simulink model "Shift_Timer_Test"  (R2023b)
settings: Solver=FixedStepDiscrete  StartTime=0.0  StopTime=160  FixedStep=0.02  RelTol=1e-3
values from neighbouring files (symbols this model uses):
  Rebuilt_Match_Time_Auto_Timer = Auto_Timer - Time_offset    (= 27)    [Shift_Timer_Test_Data.m]
  Rebuilt_Match_Time_End_Game_Timer = End_Game_Timer + Time_offset    (= 33)    [Shift_Timer_Test_Data.m]
  Rebuilt_Match_Time_Shift_1 = Time_Shift_1 - Time_offset    (= 32)    [Shift_Timer_Test_Data.m]
  Rebuilt_Match_Time_Shift_2 = Time_Shift_2 - Time_offset    (= 57)    [Shift_Timer_Test_Data.m]
  Rebuilt_Match_Time_Shift_3 = Time_Shift_3 - Time_offset    (= 82)    [Shift_Timer_Test_Data.m]
  Rebuilt_Match_Time_Shift_4 = Time_Shift_4 - Time_offset    (= 107)    [Shift_Timer_Test_Data.m]
  Rebuilt_Match_Time_Shift_Timer = Shift_Timer    (= 25)    [Shift_Timer_Test_Data.m]
undefined symbols (not defined in the file or in its folder): Rebuilt_Match_Time_Shoot_Early, Rebuilt_Match_Time_Transition, t_sample
libraries: simulink x13
settings Model: Creator=FIRSTMentor  LastModifiedBy=ander

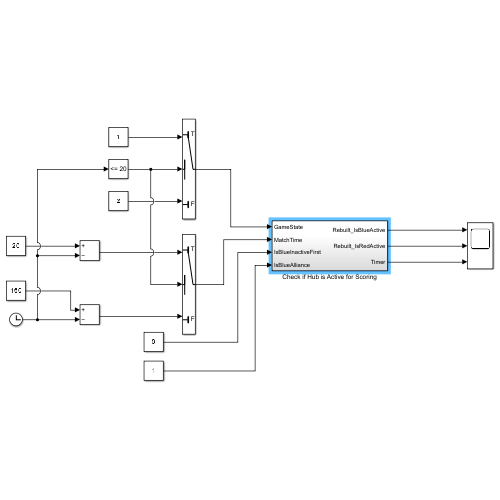
[thumbnail: Simulink's stored preview of the top-level diagram]
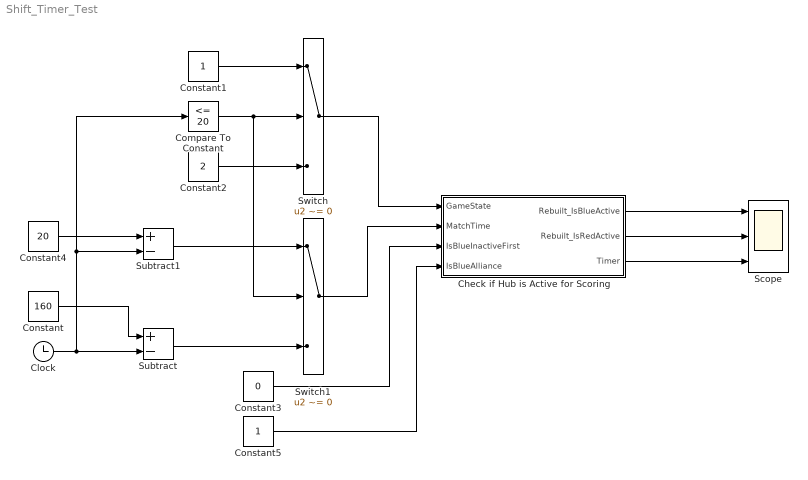
== system Shift_Timer_Test ==
  Check if Hub is Active for Scoring : Subsystem
  Clock : Clock
  Compare To Constant : simulink/Logic and Bit Operations/Compare To Constant  relop=<=  const=20  OutDataTypeStr=boolean
  Constant : Constant  Value=160
  Constant1 : Constant
  Constant2 : Constant  Value=2
  Constant3 : Constant  Value=0  OutDataTypeStr=boolean
  Constant4 : Constant  Value=20
  Constant5 : Constant  OutDataTypeStr=boolean
  Scope : Scope  NumInputPorts=3
  Subtract : Sum  Inputs=+-
  Subtract1 : Sum  Inputs=+-
  Switch : Switch  Criteria=u2 ~= 0  SaturateOnIntegerOverflow=off  InputSameDT=off
  Switch1 : Switch  Criteria=u2 ~= 0  SaturateOnIntegerOverflow=off  InputSameDT=off
  wires:
  Clock/1 -> Subtract/2, Subtract1/2, Compare To Constant/1
  Constant/1 -> Subtract/1
  Compare To Constant/1 -> Switch1/2, Switch/2
  Constant1/1 -> Switch/1
  Constant2/1 -> Switch/3
  Switch/1 -> Check if Hub is Active for Scoring/1(GameState)
  Constant3/1 -> Check if Hub is Active for Scoring/3(IsBlueInactiveFirst)
  Check if Hub is Active for Scoring/1(Rebuilt_IsBlueActive) -> Scope/1
  Check if Hub is Active for Scoring/2(Rebuilt_IsRedActive) -> Scope/2
  Check if Hub is Active for Scoring/3(Timer) -> Scope/3
  Switch1/1 -> Check if Hub is Active for Scoring/2(MatchTime)
  Subtract/1 -> Switch1/3
  Subtract1/1 -> Switch1/1
  Constant4/1 -> Subtract1/1
  Constant5/1 -> Check if Hub is Active for Scoring/4(IsBlueAlliance)

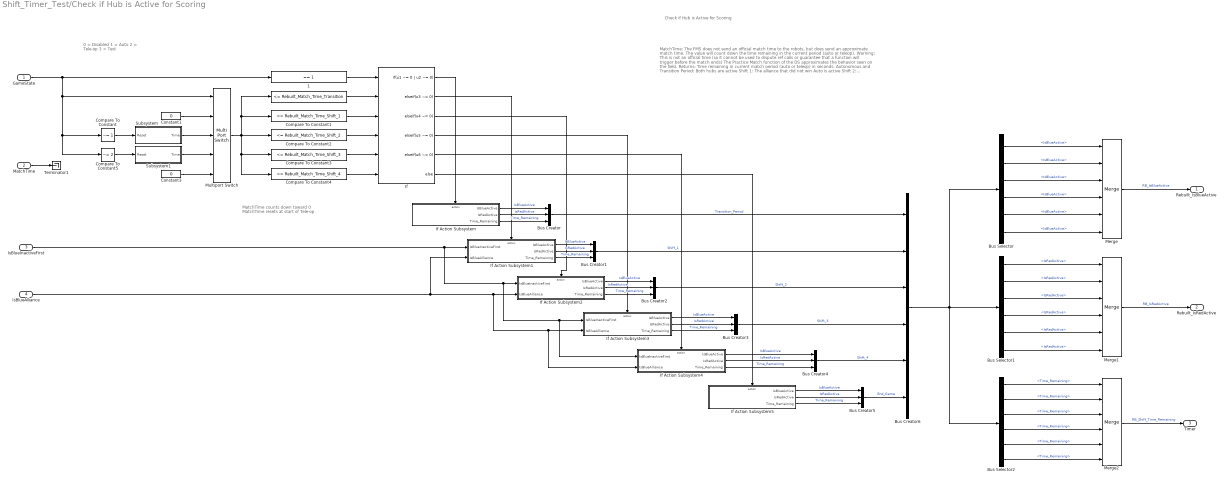
== system Shift_Timer_Test/Check if Hub is Active for Scoring ==
  note: 0 = Disabled
      | 1 = Auto
      | 2 = Tele-op
      | 3 = Test
  note: MatchTime: The FMS does not send an official match time to the robots, but does send an approximate match time. The value will count down the time remaining in the current period (auto or teleop). Warning: This is not an official time (so it cannot be used to dispute ref calls or guarantee that a function will trigger before the match ends) The Practice Match function of the DS approximates the behavior seen on the field.
      | Returns: Time remaining in current match period (auto or teleop) in seconds.
      |
      | Autonomous and Transition Period: Both hubs are active
      | Shift 1: The alliance that did not win Auto is active
      | Shift 2: Opposite of Shift 1
      | Shift 3: Same as Shift 1
      | Shift 4: Same as Shift 2
      | Endgame: Both hubs are active
  note: Check if Hub is Active for Scoring
  note: MatchTime counts down toward 0
      | MatchTime resets at start of Tele-op
  GameState : Inport
  MatchTime : Inport  Port=2
  IsBlueInactiveFirst : Inport  Port=3
  IsBlueAlliance : Inport  Port=4
  " " : simulink/Logic and Bit Operations/Compare To Constant  relop=<=  const=Rebuilt_Match_Time_Transition  OutDataTypeStr=boolean
  " 1" : simulink/Logic and Bit Operations/Compare To Constant  relop===  const=1  OutDataTypeStr=boolean
  Bus Creator{,1..5} (6 alike) : BusCreator  Inputs=3
  Bus Creator6 : BusCreator  Inputs=6
  Bus Selector : BusSelector  OutputSignals=Transition_Period.IsBlueActive,Shift_1.IsBlueActive,Shift_2.IsBlueActive,Shift_3.IsBlueActive,Shift_4.IsBlueActive,End_Game.IsBlueActive
  Bus Selector1 : BusSelector  OutputSignals=Transition_Period.IsRedActive,Shift_1.IsRedActive,Shift_2.IsRedActive,Shift_3.IsRedActive,Shift_4.IsRedActive,End_Game.IsRedActive
  Bus Selector2 : BusSelector  OutputSignals=Transition_Period.Time_Remaining,Shift_1.Time_Remaining,Shift_2.Time_Remaining,Shift_3.Time_Remaining,Shift_4.Time_Remaining,End_Game.Time_Remaining
  Compare To Constant : simulink/Logic and Bit Operations/Compare To Constant  relop=~=  const=1  OutDataTypeStr=boolean
  Compare To Constant1 : simulink/Logic and Bit Operations/Compare To Constant  relop=<=  const=Rebuilt_Match_Time_Shift_1  OutDataTypeStr=boolean
  Compare To Constant2 : simulink/Logic and Bit Operations/Compare To Constant  relop=<=  const=Rebuilt_Match_Time_Shift_2  OutDataTypeStr=boolean
  Compare To Constant3 : simulink/Logic and Bit Operations/Compare To Constant  relop=<=  const=Rebuilt_Match_Time_Shift_3  OutDataTypeStr=boolean
  Compare To Constant4 : simulink/Logic and Bit Operations/Compare To Constant  relop=<=  const=Rebuilt_Match_Time_Shift_4  OutDataTypeStr=boolean
  Compare To Constant5 : simulink/Logic and Bit Operations/Compare To Constant  relop=~=  const=2  OutDataTypeStr=boolean
  Constant1 : Constant  Value=0
  Constant3 : Constant  Value=0
  If : If  NumInputs=6  IfExpression=u1 ~= 0 | u2 ~= 0  ElseIfExpressions=u3 ~= 0,u4 ~= 0,u5 ~= 0,u6 ~= 0
  If Action Subsystem : Subsystem  TreatAsAtomicUnit=on
  If Action Subsystem1 : Subsystem  TreatAsAtomicUnit=on
  If Action Subsystem2 : Subsystem  TreatAsAtomicUnit=on
  If Action Subsystem3 : Subsystem  TreatAsAtomicUnit=on
  If Action Subsystem4 : Subsystem  TreatAsAtomicUnit=on
  If Action Subsystem5 : Subsystem  TreatAsAtomicUnit=on
  Merge : Merge  Inputs=6
  Merge1 : Merge  Inputs=6
  Merge2 : Merge  Inputs=6
  Multiport Switch : MultiPortSwitch  DataPortOrder=Zero-based contiguous  Inputs=4  zeroidx=on  SaturateOnIntegerOverflow=off  InputSameDT=off
  Subsystem : Subsystem
  Subsystem1 : Subsystem
  Terminator1 : Terminator
  Rebuilt_IsBlueActive : Outport
  Rebuilt_IsRedActive : Outport  Port=2
  Timer : Outport  Port=3
  wires:
  If/1 -> If Action Subsystem/Action
  IsBlueInactiveFirst/1 -> If Action Subsystem4/1(IsBlueInactiveFirst), If Action Subsystem3/1(IsBlueInactiveFirst), If Action Subsystem2/1(IsBlueInactiveFirst), If Action Subsystem1/1(IsBlueInactiveFirst)
  If/2 -> If Action Subsystem1/Action
  If/3 -> If Action Subsystem2/Action
  If/4 -> If Action Subsystem3/Action
  If/5 -> If Action Subsystem4/Action
  If/6 -> If Action Subsystem5/Action
  Merge/1 -> Rebuilt_IsBlueActive/1  "RB_IsBlueActive"
  Merge1/1 -> Rebuilt_IsRedActive/1  "RB_IsRedActive"
  If Action Subsystem/1(IsBlueActive) -> Bus Creator/1  "IsBlueActive"
  If Action Subsystem/2(IsRedActive) -> Bus Creator/2  "IsRedActive"
  If Action Subsystem/3(Time_Remaining) -> Bus Creator/3  "Time_Remaining"
  If Action Subsystem1/1(IsBlueActive) -> Bus Creator1/1  "IsBlueActive"
  If Action Subsystem1/2(IsRedActive) -> Bus Creator1/2  "IsRedActive"
  If Action Subsystem1/3(Time_Remaining) -> Bus Creator1/3  "Time_Remaining"
  If Action Subsystem2/1(IsBlueActive) -> Bus Creator2/1  "IsBlueActive"
  If Action Subsystem2/2(IsRedActive) -> Bus Creator2/2  "IsRedActive"
  If Action Subsystem3/1(IsBlueActive) -> Bus Creator3/1  "IsBlueActive"
  If Action Subsystem3/2(IsRedActive) -> Bus Creator3/2  "IsRedActive"
  If Action Subsystem4/1(IsBlueActive) -> Bus Creator4/1  "IsBlueActive"
  If Action Subsystem4/2(IsRedActive) -> Bus Creator4/2  "IsRedActive"
  If Action Subsystem5/1(IsBlueActive) -> Bus Creator5/1  "IsBlueActive"
  If Action Subsystem5/2(IsRedActive) -> Bus Creator5/2  "IsRedActive"
  Bus Creator/1 -> Bus Creator6/1  "Transition_Period"
  Bus Creator1/1 -> Bus Creator6/2  "Shift_1"
  Bus Creator2/1 -> Bus Creator6/3  "Shift_2"
  Bus Creator3/1 -> Bus Creator6/4  "Shift_3"
  Bus Creator4/1 -> Bus Creator6/5  "Shift_4"
  Bus Creator5/1 -> Bus Creator6/6  "End_Game"
  Bus Creator6/1 -> Bus Selector/1, Bus Selector1/1, Bus Selector2/1
  Bus Selector/1 -> Merge/1  "<IsBlueActive>"
  Bus Selector/2 -> Merge/2  "<IsBlueActive>"
  Bus Selector/3 -> Merge/3  "<IsBlueActive>"
  Bus Selector/4 -> Merge/4  "<IsBlueActive>"
  Bus Selector/5 -> Merge/5  "<IsBlueActive>"
  Bus Selector/6 -> Merge/6  "<IsBlueActive>"
  Bus Selector1/1 -> Merge1/1  "<IsRedActive>"
  Bus Selector1/2 -> Merge1/2  "<IsRedActive>"
  Bus Selector1/3 -> Merge1/3  "<IsRedActive>"
  Bus Selector1/4 -> Merge1/4  "<IsRedActive>"
  Bus Selector1/5 -> Merge1/5  "<IsRedActive>"
  Bus Selector1/6 -> Merge1/6  "<IsRedActive>"
  Bus Selector2/1 -> Merge2/1  "<Time_Remaining>"
  Bus Selector2/2 -> Merge2/2  "<Time_Remaining>"
  Bus Selector2/3 -> Merge2/3  "<Time_Remaining>"
  Bus Selector2/4 -> Merge2/4  "<Time_Remaining>"
  Bus Selector2/5 -> Merge2/5  "<Time_Remaining>"
  Bus Selector2/6 -> Merge2/6  "<Time_Remaining>"
  Merge2/1 -> Timer/1  "RB_Shift_Time_Remaining"
  If Action Subsystem2/3(Time_Remaining) -> Bus Creator2/3  "Time_Remaining"
  If Action Subsystem3/3(Time_Remaining) -> Bus Creator3/3  "Time_Remaining"
  If Action Subsystem4/3(Time_Remaining) -> Bus Creator4/3  "Time_Remaining"
  If Action Subsystem5/3(Time_Remaining) -> Bus Creator5/3  "Time_Remaining"
  " "/1 -> If/2
  Compare To Constant1/1 -> If/3
  Compare To Constant2/1 -> If/4
  Compare To Constant3/1 -> If/5
  Compare To Constant4/1 -> If/6
  " 1"/1 -> If/1
  GameState/1 -> " 1"/1, Compare To Constant5/1, Compare To Constant/1, Multiport Switch/1
  IsBlueAlliance/1 -> If Action Subsystem1/2(IsBlueAlliance), If Action Subsystem4/2(IsBlueAlliance), If Action Subsystem3/2(IsBlueAlliance), If Action Subsystem2/2(IsBlueAlliance)
  Multiport Switch/1 -> Compare To Constant2/1, Compare To Constant3/1, Compare To Constant4/1, Compare To Constant1/1, " "/1
  Constant1/1 -> Multiport Switch/2
  Constant3/1 -> Multiport Switch/5
  Subsystem/1(Time) -> Multiport Switch/3
  Compare To Constant/1 -> Subsystem/1(Reset)
  Subsystem1/1(Time) -> Multiport Switch/4
  Compare To Constant5/1 -> Subsystem1/1(Reset)
  MatchTime/1 -> Terminator1/1

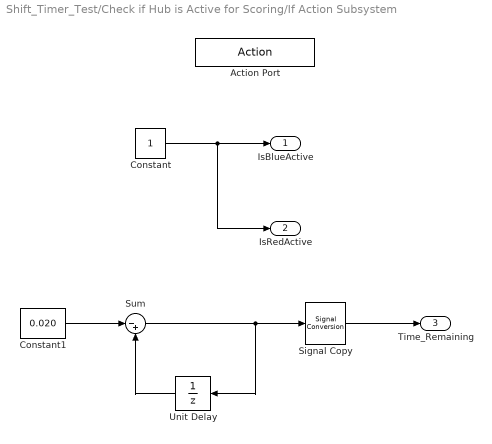
== system Shift_Timer_Test/Check if Hub is Active for Scoring/If Action Subsystem ==
  Action Port : ActionPort  InitializeStates=reset  ActionPortLabel=if(u1 ~= 0 | u2 ~= 0)
  Constant : Constant  OutDataTypeStr=boolean
  Constant1 : Constant  Value=0.020
  Signal Copy : SignalConversion  OverrideOpt=off
  Sum : Sum  Inputs=|-+
  Unit Delay : UnitDelay  InitialCondition=Rebuilt_Match_Time_Auto_Timer  SampleTime=-1  HasFrameUpgradeWarning=on
      settings: AttributesFormatString=Initial Condition = %<InitialCondition>
  IsBlueActive : Outport
  IsRedActive : Outport  Port=2
  Time_Remaining : Outport  Port=3
  wires:
  Constant/1 -> IsRedActive/1, IsBlueActive/1
  Constant1/1 -> Sum/1
  Sum/1 -> Unit Delay/1, Signal Copy/1
  Unit Delay/1 -> Sum/2
  Signal Copy/1 -> Time_Remaining/1

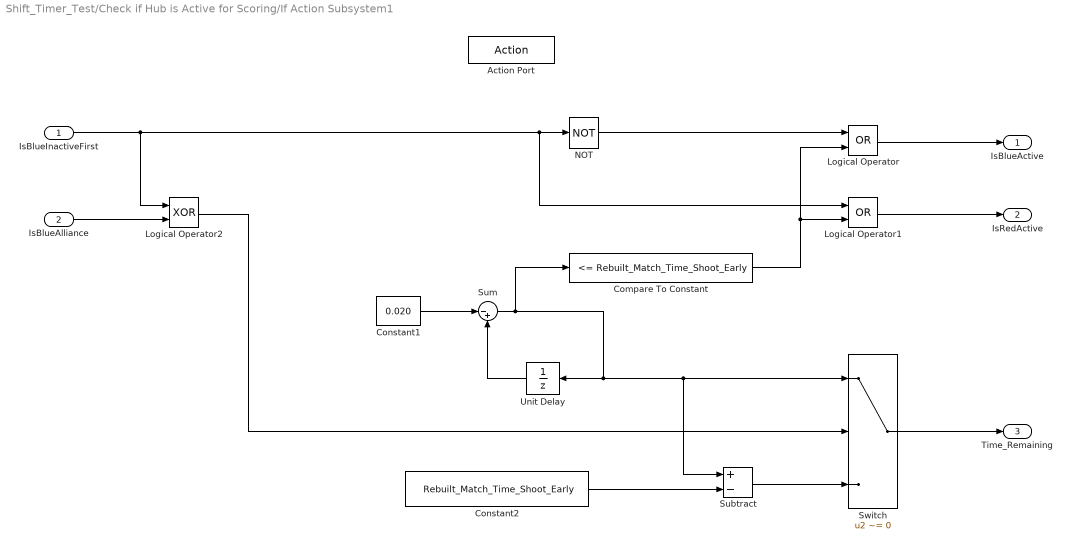
== system Shift_Timer_Test/Check if Hub is Active for Scoring/If Action Subsystem1 ==
  IsBlueInactiveFirst : Inport
  IsBlueAlliance : Inport  Port=2
  Action Port : ActionPort  ActionPortLabel=elseif(u3 ~= 0)
  Compare To Constant : simulink/Logic and Bit Operations/Compare To Constant  relop=<=  const=Rebuilt_Match_Time_Shoot_Early  OutDataTypeStr=boolean
  Constant1 : Constant  Value=0.020
  Constant2 : Constant  Value=Rebuilt_Match_Time_Shoot_Early
  Logical Operator : Logic  Operator=OR  AllPortsSameDT=off  OutDataTypeStr=boolean
  Logical Operator1 : Logic  Operator=OR  AllPortsSameDT=off  OutDataTypeStr=boolean
  Logical Operator2 : Logic  Operator=XOR  AllPortsSameDT=off  OutDataTypeStr=boolean
  NOT : Logic  Operator=NOT  AllPortsSameDT=off  OutDataTypeStr=boolean
  Subtract : Sum  Inputs=+-
  Sum : Sum  Inputs=|-+
  Switch : Switch  Criteria=u2 ~= 0  SaturateOnIntegerOverflow=off  InputSameDT=off
  Unit Delay : UnitDelay  InitialCondition=Rebuilt_Match_Time_Shift_Timer  SampleTime=-1  HasFrameUpgradeWarning=on
      settings: AttributesFormatString=Initial Condition = %<InitialCondition>
  IsBlueActive : Outport
  IsRedActive : Outport  Port=2
  Time_Remaining : Outport  Port=3
  wires:
  IsBlueInactiveFirst/1 -> Logical Operator2/1, Logical Operator1/1, NOT/1
  Constant1/1 -> Sum/1
  Unit Delay/1 -> Sum/2
  Sum/1 -> Compare To Constant/1, Subtract/1, Switch/1, Unit Delay/1
  NOT/1 -> Logical Operator/1
  Logical Operator/1 -> IsBlueActive/1
  Compare To Constant/1 -> Logical Operator1/2, Logical Operator/2
  Logical Operator1/1 -> IsRedActive/1
  IsBlueAlliance/1 -> Logical Operator2/2
  Logical Operator2/1 -> Switch/2
  Switch/1 -> Time_Remaining/1
  Subtract/1 -> Switch/3
  Constant2/1 -> Subtract/2

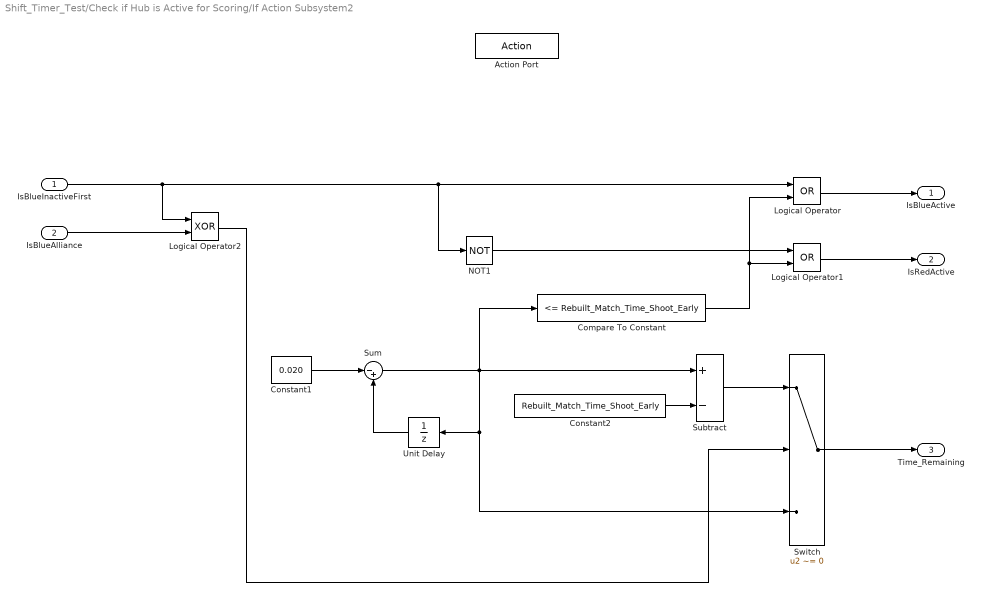
== system Shift_Timer_Test/Check if Hub is Active for Scoring/If Action Subsystem2 ==
  IsBlueInactiveFirst : Inport
  IsBlueAlliance : Inport  Port=2
  Action Port : ActionPort  ActionPortLabel=elseif(u4 ~= 0)
  Compare To Constant : simulink/Logic and Bit Operations/Compare To Constant  relop=<=  const=Rebuilt_Match_Time_Shoot_Early  OutDataTypeStr=boolean
  Constant1 : Constant  Value=0.020
  Constant2 : Constant  Value=Rebuilt_Match_Time_Shoot_Early
  Logical Operator : Logic  Operator=OR  AllPortsSameDT=off  OutDataTypeStr=boolean
  Logical Operator1 : Logic  Operator=OR  AllPortsSameDT=off  OutDataTypeStr=boolean
  Logical Operator2 : Logic  Operator=XOR  AllPortsSameDT=off  OutDataTypeStr=boolean
  NOT1 : Logic  Operator=NOT  AllPortsSameDT=off  OutDataTypeStr=boolean
  Subtract : Sum  Inputs=+-
  Sum : Sum  Inputs=|-+
  Switch : Switch  Criteria=u2 ~= 0  SaturateOnIntegerOverflow=off  InputSameDT=off
  Unit Delay : UnitDelay  InitialCondition=Rebuilt_Match_Time_Shift_Timer  SampleTime=-1  HasFrameUpgradeWarning=on
      settings: AttributesFormatString=Initial Condition = %<InitialCondition>
  IsBlueActive : Outport
  IsRedActive : Outport  Port=2
  Time_Remaining : Outport  Port=3
  wires:
  IsBlueInactiveFirst/1 -> Logical Operator2/1, NOT1/1, Logical Operator/1
  NOT1/1 -> Logical Operator1/1
  Constant1/1 -> Sum/1
  Unit Delay/1 -> Sum/2
  Sum/1 -> Switch/3, Unit Delay/1, Subtract/1, Compare To Constant/1
  Compare To Constant/1 -> Logical Operator1/2, Logical Operator/2
  Logical Operator/1 -> IsBlueActive/1
  Logical Operator1/1 -> IsRedActive/1
  Switch/1 -> Time_Remaining/1
  IsBlueAlliance/1 -> Logical Operator2/2
  Logical Operator2/1 -> Switch/2
  Subtract/1 -> Switch/1
  Constant2/1 -> Subtract/2

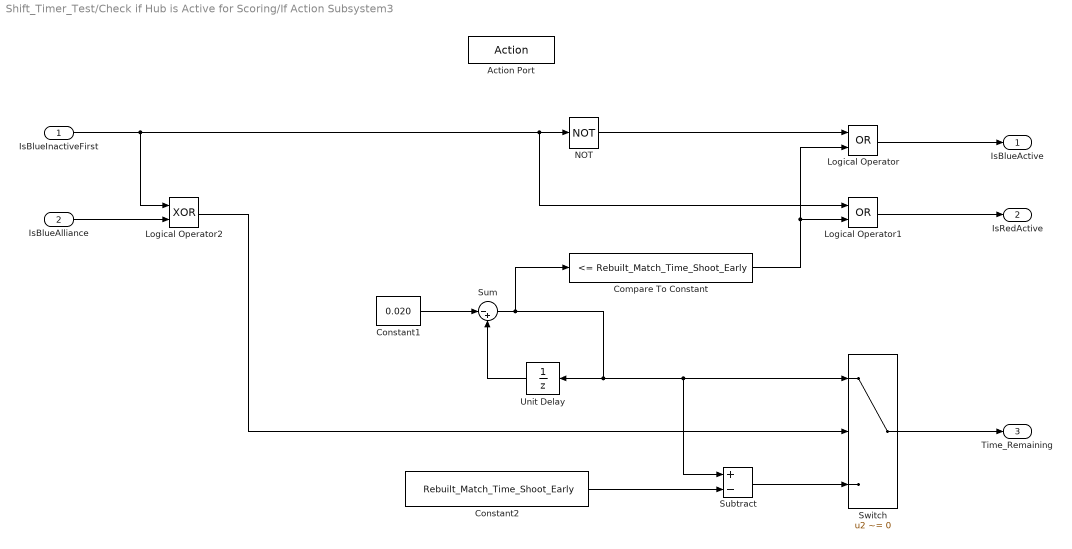
== system Shift_Timer_Test/Check if Hub is Active for Scoring/If Action Subsystem3 ==
  IsBlueInactiveFirst : Inport
  IsBlueAlliance : Inport  Port=2
  Action Port : ActionPort  ActionPortLabel=elseif(u5 ~= 0)
  Compare To Constant : simulink/Logic and Bit Operations/Compare To Constant  relop=<=  const=Rebuilt_Match_Time_Shoot_Early  OutDataTypeStr=boolean
  Constant1 : Constant  Value=0.020
  Constant2 : Constant  Value=Rebuilt_Match_Time_Shoot_Early
  Logical Operator : Logic  Operator=OR  AllPortsSameDT=off  OutDataTypeStr=boolean
  Logical Operator1 : Logic  Operator=OR  AllPortsSameDT=off  OutDataTypeStr=boolean
  Logical Operator2 : Logic  Operator=XOR  AllPortsSameDT=off  OutDataTypeStr=boolean
  NOT : Logic  Operator=NOT  AllPortsSameDT=off  OutDataTypeStr=boolean
  Subtract : Sum  Inputs=+-
  Sum : Sum  Inputs=|-+
  Switch : Switch  Criteria=u2 ~= 0  SaturateOnIntegerOverflow=off  InputSameDT=off
  Unit Delay : UnitDelay  InitialCondition=Rebuilt_Match_Time_Shift_Timer  SampleTime=-1  HasFrameUpgradeWarning=on
      settings: AttributesFormatString=Initial Condition = %<InitialCondition>
  IsBlueActive : Outport
  IsRedActive : Outport  Port=2
  Time_Remaining : Outport  Port=3
  wires:
  Constant2/1 -> Subtract/2
  Subtract/1 -> Switch/3
  Switch/1 -> Time_Remaining/1
  Logical Operator2/1 -> Switch/2
  IsBlueAlliance/1 -> Logical Operator2/2
  Logical Operator1/1 -> IsRedActive/1
  Compare To Constant/1 -> Logical Operator/2, Logical Operator1/2
  Logical Operator/1 -> IsBlueActive/1
  NOT/1 -> Logical Operator/1
  Sum/1 -> Unit Delay/1, Switch/1, Subtract/1, Compare To Constant/1
  Unit Delay/1 -> Sum/2
  Constant1/1 -> Sum/1
  IsBlueInactiveFirst/1 -> NOT/1, Logical Operator1/1, Logical Operator2/1

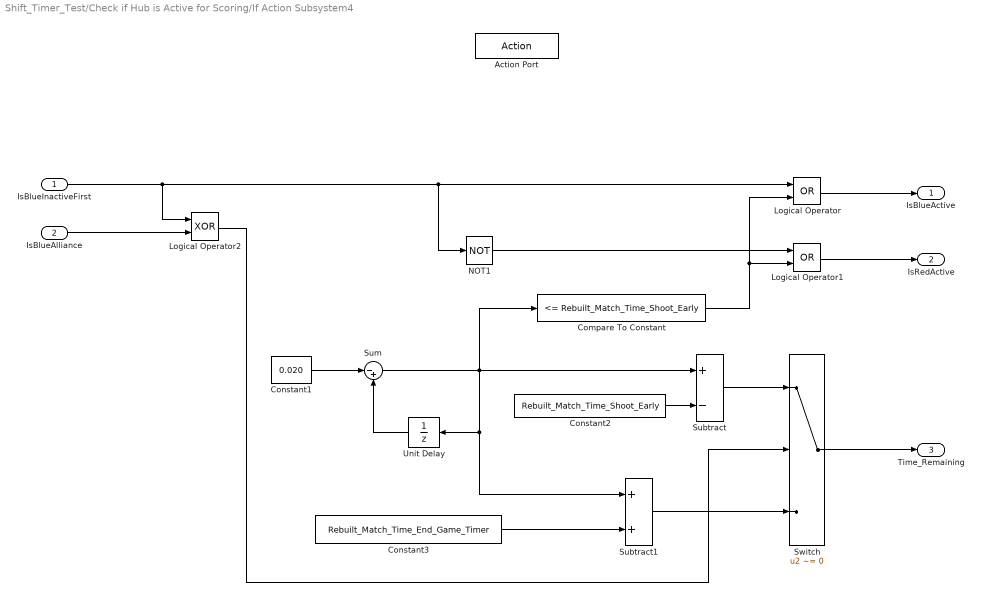
== system Shift_Timer_Test/Check if Hub is Active for Scoring/If Action Subsystem4 ==
  IsBlueInactiveFirst : Inport
  IsBlueAlliance : Inport  Port=2
  Action Port : ActionPort  ActionPortLabel=elseif(u6 ~= 0)
  Compare To Constant : simulink/Logic and Bit Operations/Compare To Constant  relop=<=  const=Rebuilt_Match_Time_Shoot_Early  OutDataTypeStr=boolean
  Constant1 : Constant  Value=0.020
  Constant2 : Constant  Value=Rebuilt_Match_Time_Shoot_Early
  Constant3 : Constant  Value=Rebuilt_Match_Time_End_Game_Timer
  Logical Operator : Logic  Operator=OR  AllPortsSameDT=off  OutDataTypeStr=boolean
  Logical Operator1 : Logic  Operator=OR  AllPortsSameDT=off  OutDataTypeStr=boolean
  Logical Operator2 : Logic  Operator=XOR  AllPortsSameDT=off  OutDataTypeStr=boolean
  NOT1 : Logic  Operator=NOT  AllPortsSameDT=off  OutDataTypeStr=boolean
  Subtract : Sum  Inputs=+-
  Subtract1 : Sum
  Sum : Sum  Inputs=|-+
  Switch : Switch  Criteria=u2 ~= 0  SaturateOnIntegerOverflow=off  InputSameDT=off
  Unit Delay : UnitDelay  InitialCondition=Rebuilt_Match_Time_Shift_Timer  SampleTime=-1  HasFrameUpgradeWarning=on
      settings: AttributesFormatString=Initial Condition = %<InitialCondition>
  IsBlueActive : Outport
  IsRedActive : Outport  Port=2
  Time_Remaining : Outport  Port=3
  wires:
  Constant2/1 -> Subtract/2
  Subtract/1 -> Switch/1
  Logical Operator2/1 -> Switch/2
  IsBlueAlliance/1 -> Logical Operator2/2
  Switch/1 -> Time_Remaining/1
  Logical Operator1/1 -> IsRedActive/1
  Logical Operator/1 -> IsBlueActive/1
  Compare To Constant/1 -> Logical Operator/2, Logical Operator1/2
  Sum/1 -> Compare To Constant/1, Subtract/1, Subtract1/1, Unit Delay/1
  Unit Delay/1 -> Sum/2
  Constant1/1 -> Sum/1
  NOT1/1 -> Logical Operator1/1
  IsBlueInactiveFirst/1 -> Logical Operator/1, NOT1/1, Logical Operator2/1
  Subtract1/1 -> Switch/3
  Constant3/1 -> Subtract1/2

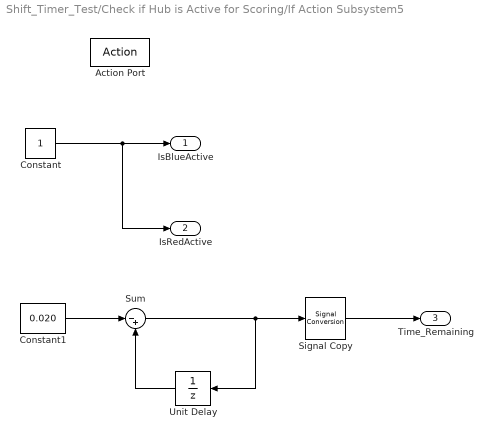
== system Shift_Timer_Test/Check if Hub is Active for Scoring/If Action Subsystem5 ==
  Action Port : ActionPort  ActionPortLabel=else
  Constant : Constant  OutDataTypeStr=boolean
  Constant1 : Constant  Value=0.020
  Signal Copy : SignalConversion  OverrideOpt=off
  Sum : Sum  Inputs=|-+
  Unit Delay : UnitDelay  InitialCondition=Rebuilt_Match_Time_End_Game_Timer  SampleTime=-1  HasFrameUpgradeWarning=on
      settings: AttributesFormatString=Initial Condition = %<InitialCondition>
  IsBlueActive : Outport
  IsRedActive : Outport  Port=2
  Time_Remaining : Outport  Port=3
  wires:
  Constant/1 -> IsBlueActive/1, IsRedActive/1
  Constant1/1 -> Sum/1
  Signal Copy/1 -> Time_Remaining/1
  Unit Delay/1 -> Sum/2
  Sum/1 -> Unit Delay/1, Signal Copy/1

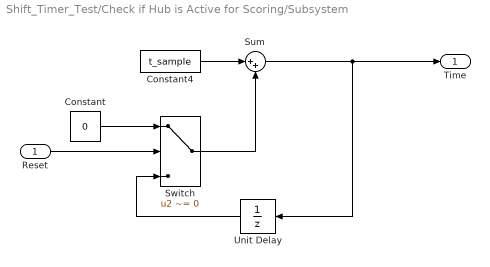
== system Shift_Timer_Test/Check if Hub is Active for Scoring/Subsystem ==
  Reset : Inport
  Constant : Constant  Value=0
  Constant4 : Constant  Value=t_sample
  Sum : Sum  Inputs=|++
  Switch : Switch  Criteria=u2 ~= 0  SaturateOnIntegerOverflow=off  InputSameDT=off
  Unit Delay : UnitDelay  SampleTime=-1  HasFrameUpgradeWarning=on
  Time : Outport
  wires:
  Constant4/1 -> Sum/1
  Sum/1 -> Unit Delay/1, Time/1
  Reset/1 -> Switch/2
  Constant/1 -> Switch/1
  Switch/1 -> Sum/2
  Unit Delay/1 -> Switch/3

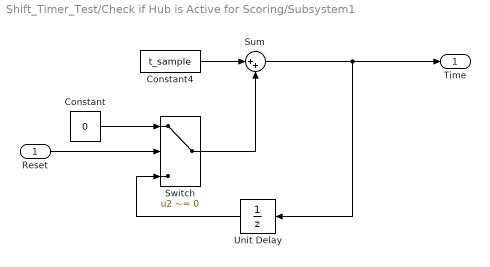
== system Shift_Timer_Test/Check if Hub is Active for Scoring/Subsystem1 ==
  Reset : Inport
  Constant : Constant  Value=0
  Constant4 : Constant  Value=t_sample
  Sum : Sum  Inputs=|++
  Switch : Switch  Criteria=u2 ~= 0  SaturateOnIntegerOverflow=off  InputSameDT=off
  Unit Delay : UnitDelay  SampleTime=-1  HasFrameUpgradeWarning=on
  Time : Outport
  wires:
  Unit Delay/1 -> Switch/3
  Switch/1 -> Sum/2
  Constant/1 -> Switch/1
  Reset/1 -> Switch/2
  Sum/1 -> Time/1, Unit Delay/1
  Constant4/1 -> Sum/1
